simulink model "Bramki_zad1_4"  (R2025a)
settings: Solver=VariableStepAuto  StopTime=inf
libraries: visiontextngfix x1
settings Model: Creator=PM  LastModifiedBy=ai
settings SFSimCC: SimGPUStackLimitPerThread=51200  SimGPUMallocThreshold=200
settings RTWCC: GPUStackLimitPerThread=51200  GPUMallocThreshold=200

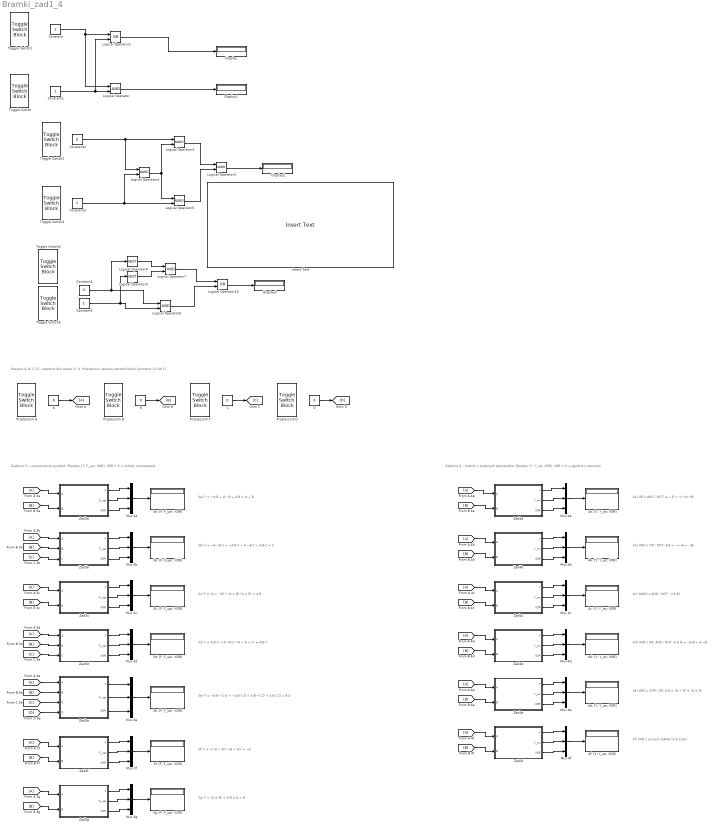
== system Bramki_zad1_4 ==
  note: Wejścia A, B, C, D – wspólne dla zadań 3 i 4. Przełącznik ustawia wartość bloku Constant (0 lub 1).
  note: 3a) F = ¬A·B + A·¬B + A·B = A + B
  note: 3b) F = ¬A·¬B·C + ¬A·B·C + A·¬B·C + A·B·C = C
  note: 3c) F = (A + ¬B)·(¬A + B)·(A + B) = A·B
  note: 3d) F = A·B·C·¬(A·¬B·C)·(A + B + C) = A·B·C
  note: 3e) F = ¬A·B·¬C·D + ¬A·B·C·D + A·B·¬C·D + A·B·C·D = B·D
  note: 3f) F = ¬((A + B)·(¬B + A)) = ¬A
  note: 3g) F = (A ⊕ B) + A·B = A + B
  note: 4a) OR z AND i NOT: A + B = ¬(¬A·¬B)
  note: 4b) AND z OR i NOT: A·B = ¬(¬A + ¬B)
  note: 4c) NAND z AND i NOT: ¬(A·B)
  note: 4d) XOR z OR, AND i NOT: A ⊕ B = ¬A·B + A·¬B
  note: 4e) AND z XOR i OR: A·B = (A + B) ⊕ (A ⊕ B)
  note: 4f) XOR z samych NAND (4 bramki)
  note: Zadanie 3 – upraszczanie wyrażeń. Display: [F; F_upr; XOR], XOR = 0 → układy równoważne
  note: Zadanie 4 – bramki z podanych elementów. Display: [Y; Y_wz; XOR], XOR = 0 → zgodne z wzorcem
  3a: [F; F_upr; XOR] : Display
  3b: [F; F_upr; XOR] : Display
  3c: [F; F_upr; XOR] : Display
  3d: [F; F_upr; XOR] : Display
  3e: [F; F_upr; XOR] : Display
  3f: [F; F_upr; XOR] : Display
  3g: [F; F_upr; XOR] : Display
  4a: [Y; Y_wz; XOR] : Display
  4b: [Y; Y_wz; XOR] : Display
  4c: [Y; Y_wz; XOR] : Display
  4d: [Y; Y_wz; XOR] : Display
  4e: [Y; Y_wz; XOR] : Display
  4f: [Y; Y_wz; XOR] : Display
  A : Constant  Value=0  OutDataTypeStr=boolean  SampleTime=0.1
  B : Constant  Value=0  OutDataTypeStr=boolean  SampleTime=0.1
  C : Constant  Value=0  OutDataTypeStr=boolean  SampleTime=0.1
  Constant{,1,3,5} (4 alike) : Constant
  Constant2 : Constant  Value=0
  Constant4 : Constant  Value=0
  D : Constant  Value=0  OutDataTypeStr=boolean  SampleTime=0.1
  Display{,1..3} (4 alike) : Display
  From A 3a : From
  From A 3b : From
  From A 3c : From
  From A 3d : From
  From A 3e : From
  From A 3f : From
  From A 3g : From
  From A 4a : From
  From A 4b : From
  From A 4c : From
  From A 4d : From
  From A 4e : From
  From A 4f : From
  Goto A : Goto
  Insert Text : visiontextngfix/Insert Text  inputType=Obsolete  theText='TO JEST TO SAMO wooooooooow'  getTextLocFrom=Specify via dialog  textLoc=[1 1]  getTextColorFrom=Specify via dialog  textColor=[0 0 0]  getTextIntensityFrom=Specify via dialog  textIntensity=0  getTextOpacityFrom=Specify via dialog  textOpacity=1.0  dummyVar2=0  dummyVar3=0  dummyVar4=0  imagePorts=One multidimensional signal  isInputTransposed=off  fontFace=LucidaSansRegular  dummyVar1=0  blockFontSize=12  antiAliased=on
  Logical Operator : Logic  AllPortsSameDT=off  OutDataTypeStr=boolean
  Logical Operator1 : Logic  Operator=OR  AllPortsSameDT=off  OutDataTypeStr=boolean
  Logical Operator10 : Logic  Operator=OR  AllPortsSameDT=off  OutDataTypeStr=boolean
  Logical Operator{2..5} (4 alike) : Logic  Operator=NAND  AllPortsSameDT=off  OutDataTypeStr=boolean
  Logical Operator6 : Logic  AllPortsSameDT=off  OutDataTypeStr=boolean
  Logical Operator7 : Logic  AllPortsSameDT=off  OutDataTypeStr=boolean
  Logical Operator8 : Logic  Operator=NOT  AllPortsSameDT=off  OutDataTypeStr=boolean
  Logical Operator9 : Logic  Operator=NOT  AllPortsSameDT=off  OutDataTypeStr=boolean
  Mux 3a : Mux  Inputs=3
  Mux 3b : Mux  Inputs=3
  Mux 3c : Mux  Inputs=3
  Mux 3d : Mux  Inputs=3
  Mux 3e : Mux  Inputs=3
  Mux 3f : Mux  Inputs=3
  Mux 3g : Mux  Inputs=3
  Mux 4a : Mux  Inputs=3
  Mux 4b : Mux  Inputs=3
  Mux 4c : Mux  Inputs=3
  Mux 4d : Mux  Inputs=3
  Mux 4e : Mux  Inputs=3
  Mux 4f : Mux  Inputs=3
  Przelacznik A : ToggleSwitchBlock
  Przelacznik B : ToggleSwitchBlock
  Przelacznik C : ToggleSwitchBlock
  Przelacznik D : ToggleSwitchBlock
  Toggle Switch{,1..5} (6 alike) : ToggleSwitchBlock
  Zad3a : Subsystem
  Zad3b : Subsystem
  Zad3c : Subsystem
  Zad3d : Subsystem
  Zad3e : Subsystem
  Zad3f : Subsystem
  Zad3g : Subsystem
  Zad4a : Subsystem
  Zad4b : Subsystem
  Zad4c : Subsystem
  Zad4d : Subsystem
  Zad4e : Subsystem
  Zad4f : Subsystem
  wires:
  Constant/1 -> Logical Operator/1, Logical Operator1/1
  Constant1/1 -> Logical Operator/2, Logical Operator1/2
  Logical Operator1/1 -> Display/1
  Logical Operator/1 -> Display1/1
  Logical Operator2/1 -> Logical Operator3/1
  Logical Operator5/1 -> Logical Operator3/2
  Logical Operator4/1 -> Logical Operator5/1, Logical Operator2/2
  Constant2/1 -> Logical Operator4/1, Logical Operator2/1
  Constant3/1 -> Logical Operator4/2, Logical Operator5/2
  Logical Operator3/1 -> Display2/1
  Logical Operator7/1 -> Logical Operator10/1
  Logical Operator6/1 -> Logical Operator10/2
  Logical Operator10/1 -> Display3/1
  Logical Operator8/1 -> Logical Operator7/1
  Logical Operator9/1 -> Logical Operator7/2
  Constant5/1 -> Logical Operator9/1, Logical Operator6/2
  Constant4/1 -> Logical Operator8/1, Logical Operator6/1
  A/1 -> Goto A/1
  B/1 -> [B]
  C/1 -> [C]
  D/1 -> [D]
  From A 3a/1 -> Zad3a/1(A)
  [B] -> Zad3a/2(B)
  Zad3a/1(F) -> Mux 3a/1
  Zad3a/2(F_upr) -> Mux 3a/2
  Zad3a/3(XOR) -> Mux 3a/3
  Mux 3a/1 -> 3a: [F; F_upr; XOR]/1
  From A 3b/1 -> Zad3b/1(A)
  [B] -> Zad3b/2(B)
  [C] -> Zad3b/3(C)
  Zad3b/1(F) -> Mux 3b/1
  Zad3b/2(F_upr) -> Mux 3b/2
  Zad3b/3(XOR) -> Mux 3b/3
  Mux 3b/1 -> 3b: [F; F_upr; XOR]/1
  From A 3c/1 -> Zad3c/1(A)
  [B] -> Zad3c/2(B)
  Zad3c/1(F) -> Mux 3c/1
  Zad3c/2(F_upr) -> Mux 3c/2
  Zad3c/3(XOR) -> Mux 3c/3
  Mux 3c/1 -> 3c: [F; F_upr; XOR]/1
  From A 3d/1 -> Zad3d/1(A)
  [B] -> Zad3d/2(B)
  [C] -> Zad3d/3(C)
  Zad3d/1(F) -> Mux 3d/1
  Zad3d/2(F_upr) -> Mux 3d/2
  Zad3d/3(XOR) -> Mux 3d/3
  Mux 3d/1 -> 3d: [F; F_upr; XOR]/1
  From A 3e/1 -> Zad3e/1(A)
  [B] -> Zad3e/2(B)
  [C] -> Zad3e/3(C)
  [D] -> Zad3e/4(D)
  Zad3e/1(F) -> Mux 3e/1
  Zad3e/2(F_upr) -> Mux 3e/2
  Zad3e/3(XOR) -> Mux 3e/3
  Mux 3e/1 -> 3e: [F; F_upr; XOR]/1
  From A 3f/1 -> Zad3f/1(A)
  [B] -> Zad3f/2(B)
  Zad3f/1(F) -> Mux 3f/1
  Zad3f/2(F_upr) -> Mux 3f/2
  Zad3f/3(XOR) -> Mux 3f/3
  Mux 3f/1 -> 3f: [F; F_upr; XOR]/1
  From A 3g/1 -> Zad3g/1(A)
  [B] -> Zad3g/2(B)
  Zad3g/1(F) -> Mux 3g/1
  Zad3g/2(F_upr) -> Mux 3g/2
  Zad3g/3(XOR) -> Mux 3g/3
  Mux 3g/1 -> 3g: [F; F_upr; XOR]/1
  From A 4a/1 -> Zad4a/1(A)
  [B] -> Zad4a/2(B)
  Zad4a/1(Y) -> Mux 4a/1
  Zad4a/2(Y_wz) -> Mux 4a/2
  Zad4a/3(XOR) -> Mux 4a/3
  Mux 4a/1 -> 4a: [Y; Y_wz; XOR]/1
  From A 4b/1 -> Zad4b/1(A)
  [B] -> Zad4b/2(B)
  Zad4b/1(Y) -> Mux 4b/1
  Zad4b/2(Y_wz) -> Mux 4b/2
  Zad4b/3(XOR) -> Mux 4b/3
  Mux 4b/1 -> 4b: [Y; Y_wz; XOR]/1
  From A 4c/1 -> Zad4c/1(A)
  [B] -> Zad4c/2(B)
  Zad4c/1(Y) -> Mux 4c/1
  Zad4c/2(Y_wz) -> Mux 4c/2
  Zad4c/3(XOR) -> Mux 4c/3
  Mux 4c/1 -> 4c: [Y; Y_wz; XOR]/1
  From A 4d/1 -> Zad4d/1(A)
  [B] -> Zad4d/2(B)
  Zad4d/1(Y) -> Mux 4d/1
  Zad4d/2(Y_wz) -> Mux 4d/2
  Zad4d/3(XOR) -> Mux 4d/3
  Mux 4d/1 -> 4d: [Y; Y_wz; XOR]/1
  From A 4e/1 -> Zad4e/1(A)
  [B] -> Zad4e/2(B)
  Zad4e/1(Y) -> Mux 4e/1
  Zad4e/2(Y_wz) -> Mux 4e/2
  Zad4e/3(XOR) -> Mux 4e/3
  Mux 4e/1 -> 4e: [Y; Y_wz; XOR]/1
  From A 4f/1 -> Zad4f/1(A)
  [B] -> Zad4f/2(B)
  Zad4f/1(Y) -> Mux 4f/1
  Zad4f/2(Y_wz) -> Mux 4f/2
  Zad4f/3(XOR) -> Mux 4f/3
  Mux 4f/1 -> 4f: [Y; Y_wz; XOR]/1

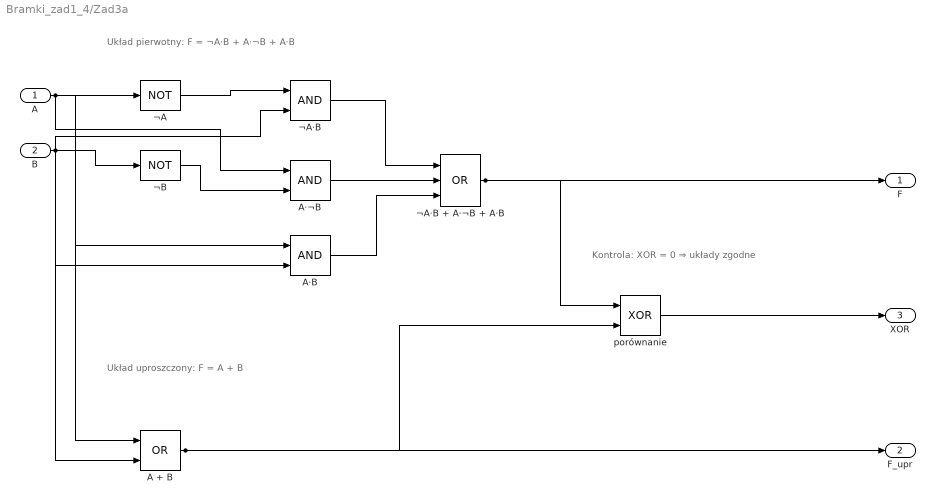
== system Bramki_zad1_4/Zad3a ==
  note: Układ pierwotny: F = ¬A·B + A·¬B + A·B
  note: Układ uproszczony: F = A + B
  note: Kontrola: XOR = 0 ⇒ układy zgodne
  A : Inport
  B : Inport  Port=2
  A + B : Logic  Operator=OR  IconShape=distinctive  AllPortsSameDT=off  OutDataTypeStr=boolean
  A·B : Logic  IconShape=distinctive  AllPortsSameDT=off  OutDataTypeStr=boolean
  A·¬B : Logic  IconShape=distinctive  AllPortsSameDT=off  OutDataTypeStr=boolean
  porównanie : Logic  Operator=XOR  IconShape=distinctive  AllPortsSameDT=off  OutDataTypeStr=boolean
  ¬A : Logic  Operator=NOT  Inputs=1  IconShape=distinctive  AllPortsSameDT=off  OutDataTypeStr=boolean
  ¬A·B : Logic  IconShape=distinctive  AllPortsSameDT=off  OutDataTypeStr=boolean
  ¬A·B + A·¬B + A·B : Logic  Operator=OR  Inputs=3  IconShape=distinctive  AllPortsSameDT=off  OutDataTypeStr=boolean
  ¬B : Logic  Operator=NOT  Inputs=1  IconShape=distinctive  AllPortsSameDT=off  OutDataTypeStr=boolean
  F : Outport
  F_upr : Outport  Port=2
  XOR : Outport  Port=3
  wires:
  A/1 -> ¬A/1, A·¬B/1, A·B/1, A + B/1
  B/1 -> ¬B/1, ¬A·B/2, A·B/2, A + B/2
  ¬A/1 -> ¬A·B/1
  ¬B/1 -> A·¬B/2
  ¬A·B/1 -> ¬A·B + A·¬B + A·B/1
  A·¬B/1 -> ¬A·B + A·¬B + A·B/2
  A·B/1 -> ¬A·B + A·¬B + A·B/3
  ¬A·B + A·¬B + A·B/1 -> porównanie/1, F/1
  A + B/1 -> porównanie/2, F_upr/1
  porównanie/1 -> XOR/1

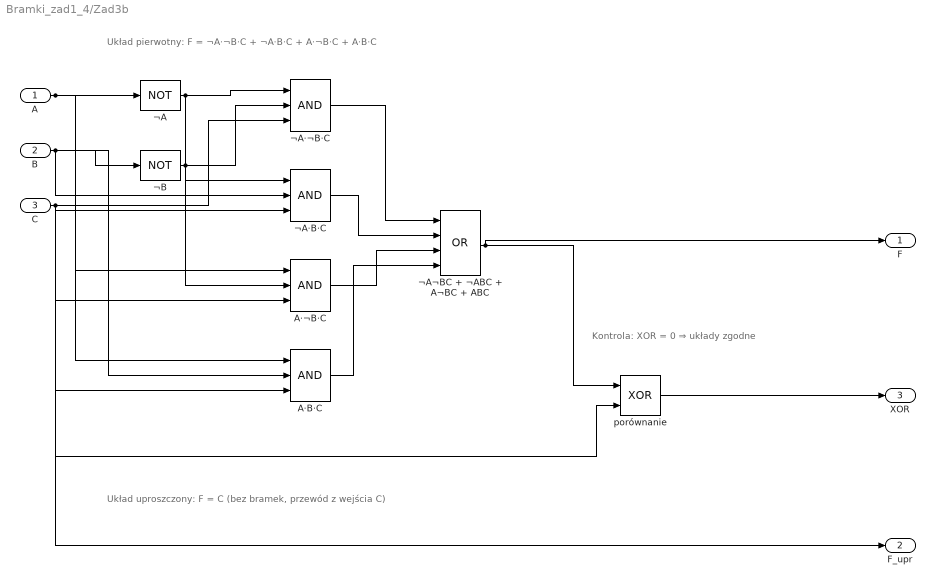
== system Bramki_zad1_4/Zad3b ==
  note: Układ pierwotny: F = ¬A·¬B·C + ¬A·B·C + A·¬B·C + A·B·C
  note: Układ uproszczony: F = C (bez bramek, przewód z wejścia C)
  note: Kontrola: XOR = 0 ⇒ układy zgodne
  A : Inport
  B : Inport  Port=2
  C : Inport  Port=3
  A·B·C : Logic  Inputs=3  IconShape=distinctive  AllPortsSameDT=off  OutDataTypeStr=boolean
  A·¬B·C : Logic  Inputs=3  IconShape=distinctive  AllPortsSameDT=off  OutDataTypeStr=boolean
  porównanie : Logic  Operator=XOR  IconShape=distinctive  AllPortsSameDT=off  OutDataTypeStr=boolean
  ¬A : Logic  Operator=NOT  Inputs=1  IconShape=distinctive  AllPortsSameDT=off  OutDataTypeStr=boolean
  ¬A¬BC + ¬ABC + A¬BC + ABC : Logic  Operator=OR  Inputs=4  IconShape=distinctive  AllPortsSameDT=off  OutDataTypeStr=boolean
  ¬A·B·C : Logic  Inputs=3  IconShape=distinctive  AllPortsSameDT=off  OutDataTypeStr=boolean
  ¬A·¬B·C : Logic  Inputs=3  IconShape=distinctive  AllPortsSameDT=off  OutDataTypeStr=boolean
  ¬B : Logic  Operator=NOT  Inputs=1  IconShape=distinctive  AllPortsSameDT=off  OutDataTypeStr=boolean
  F : Outport
  F_upr : Outport  Port=2
  XOR : Outport  Port=3
  wires:
  A/1 -> ¬A/1, A·¬B·C/1, A·B·C/1
  B/1 -> ¬B/1, ¬A·B·C/2, A·B·C/2
  ¬A/1 -> ¬A·¬B·C/1, ¬A·B·C/1
  ¬B/1 -> ¬A·¬B·C/2, A·¬B·C/2
  C/1 -> ¬A·¬B·C/3, ¬A·B·C/3, A·¬B·C/3, A·B·C/3, porównanie/2, F_upr/1
  ¬A·¬B·C/1 -> ¬A¬BC + ¬ABC + A¬BC + ABC/1
  ¬A·B·C/1 -> ¬A¬BC + ¬ABC + A¬BC + ABC/2
  A·¬B·C/1 -> ¬A¬BC + ¬ABC + A¬BC + ABC/3
  A·B·C/1 -> ¬A¬BC + ¬ABC + A¬BC + ABC/4
  ¬A¬BC + ¬ABC + A¬BC + ABC/1 -> porównanie/1, F/1
  porównanie/1 -> XOR/1

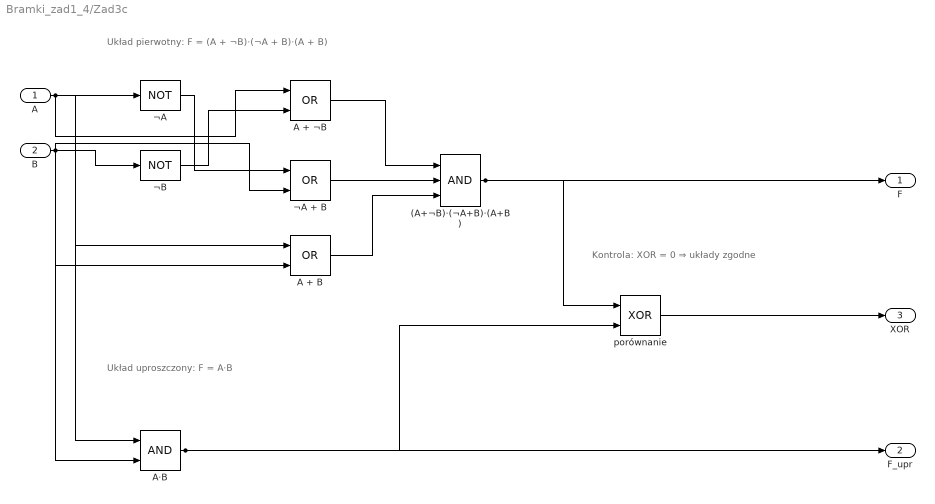
== system Bramki_zad1_4/Zad3c ==
  note: Układ pierwotny: F = (A + ¬B)·(¬A + B)·(A + B)
  note: Układ uproszczony: F = A·B
  note: Kontrola: XOR = 0 ⇒ układy zgodne
  A : Inport
  B : Inport  Port=2
  (A+¬B)·(¬A+B)·(A+B) : Logic  Inputs=3  IconShape=distinctive  AllPortsSameDT=off  OutDataTypeStr=boolean
  A + B : Logic  Operator=OR  IconShape=distinctive  AllPortsSameDT=off  OutDataTypeStr=boolean
  A + ¬B : Logic  Operator=OR  IconShape=distinctive  AllPortsSameDT=off  OutDataTypeStr=boolean
  A·B : Logic  IconShape=distinctive  AllPortsSameDT=off  OutDataTypeStr=boolean
  porównanie : Logic  Operator=XOR  IconShape=distinctive  AllPortsSameDT=off  OutDataTypeStr=boolean
  ¬A : Logic  Operator=NOT  Inputs=1  IconShape=distinctive  AllPortsSameDT=off  OutDataTypeStr=boolean
  ¬A + B : Logic  Operator=OR  IconShape=distinctive  AllPortsSameDT=off  OutDataTypeStr=boolean
  ¬B : Logic  Operator=NOT  Inputs=1  IconShape=distinctive  AllPortsSameDT=off  OutDataTypeStr=boolean
  F : Outport
  F_upr : Outport  Port=2
  XOR : Outport  Port=3
  wires:
  A/1 -> ¬A/1, A + ¬B/1, A + B/1, A·B/1
  B/1 -> ¬B/1, ¬A + B/2, A + B/2, A·B/2
  ¬B/1 -> A + ¬B/2
  ¬A/1 -> ¬A + B/1
  A + ¬B/1 -> (A+¬B)·(¬A+B)·(A+B)/1
  ¬A + B/1 -> (A+¬B)·(¬A+B)·(A+B)/2
  A + B/1 -> (A+¬B)·(¬A+B)·(A+B)/3
  (A+¬B)·(¬A+B)·(A+B)/1 -> porównanie/1, F/1
  A·B/1 -> porównanie/2, F_upr/1
  porównanie/1 -> XOR/1

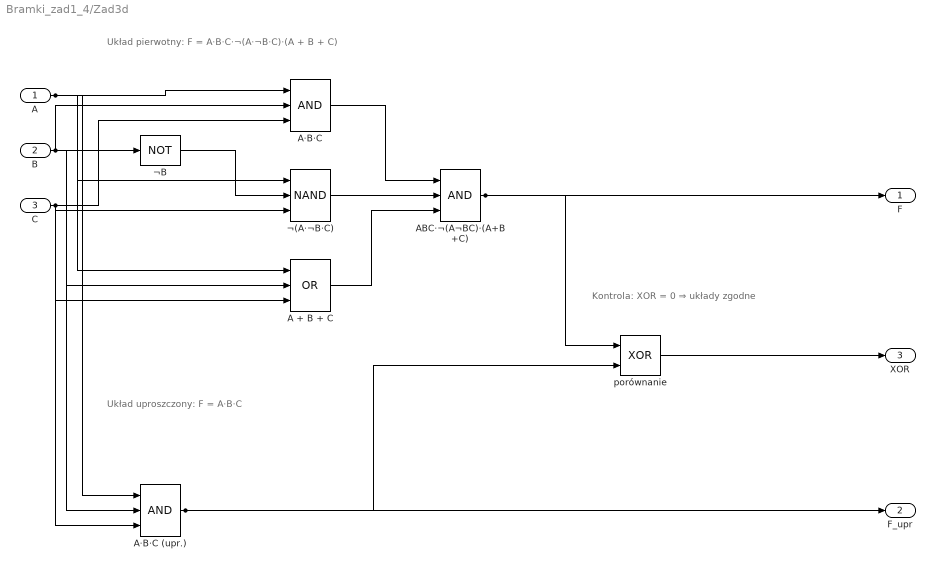
== system Bramki_zad1_4/Zad3d ==
  note: Układ pierwotny: F = A·B·C·¬(A·¬B·C)·(A + B + C)
  note: Układ uproszczony: F = A·B·C
  note: Kontrola: XOR = 0 ⇒ układy zgodne
  A : Inport
  B : Inport  Port=2
  C : Inport  Port=3
  A + B + C : Logic  Operator=OR  Inputs=3  IconShape=distinctive  AllPortsSameDT=off  OutDataTypeStr=boolean
  ABC·¬(A¬BC)·(A+B+C) : Logic  Inputs=3  IconShape=distinctive  AllPortsSameDT=off  OutDataTypeStr=boolean
  A·B·C : Logic  Inputs=3  IconShape=distinctive  AllPortsSameDT=off  OutDataTypeStr=boolean
  A·B·C (upr.) : Logic  Inputs=3  IconShape=distinctive  AllPortsSameDT=off  OutDataTypeStr=boolean
  porównanie : Logic  Operator=XOR  IconShape=distinctive  AllPortsSameDT=off  OutDataTypeStr=boolean
  ¬(A·¬B·C) : Logic  Operator=NAND  Inputs=3  IconShape=distinctive  AllPortsSameDT=off  OutDataTypeStr=boolean
  ¬B : Logic  Operator=NOT  Inputs=1  IconShape=distinctive  AllPortsSameDT=off  OutDataTypeStr=boolean
  F : Outport
  F_upr : Outport  Port=2
  XOR : Outport  Port=3
  wires:
  B/1 -> ¬B/1, A·B·C/2, A + B + C/2, A·B·C (upr.)/2
  A/1 -> A·B·C/1, ¬(A·¬B·C)/1, A + B + C/1, A·B·C (upr.)/1
  C/1 -> A·B·C/3, ¬(A·¬B·C)/3, A + B + C/3, A·B·C (upr.)/3
  ¬B/1 -> ¬(A·¬B·C)/2
  A·B·C/1 -> ABC·¬(A¬BC)·(A+B+C)/1
  ¬(A·¬B·C)/1 -> ABC·¬(A¬BC)·(A+B+C)/2
  A + B + C/1 -> ABC·¬(A¬BC)·(A+B+C)/3
  ABC·¬(A¬BC)·(A+B+C)/1 -> porównanie/1, F/1
  A·B·C (upr.)/1 -> porównanie/2, F_upr/1
  porównanie/1 -> XOR/1

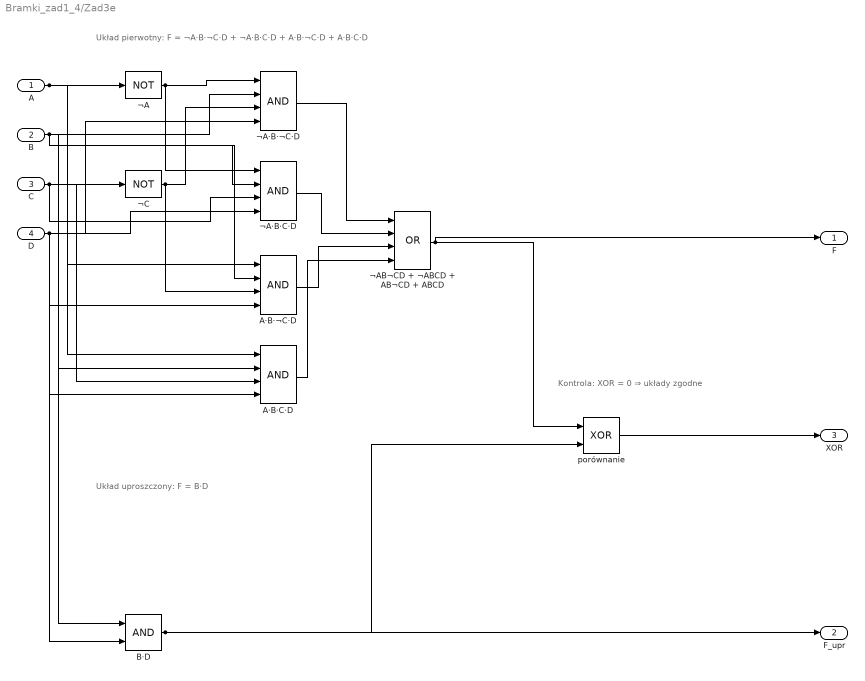
== system Bramki_zad1_4/Zad3e ==
  note: Układ pierwotny: F = ¬A·B·¬C·D + ¬A·B·C·D + A·B·¬C·D + A·B·C·D
  note: Układ uproszczony: F = B·D
  note: Kontrola: XOR = 0 ⇒ układy zgodne
  A : Inport
  B : Inport  Port=2
  C : Inport  Port=3
  D : Inport  Port=4
  A·B·C·D : Logic  Inputs=4  IconShape=distinctive  AllPortsSameDT=off  OutDataTypeStr=boolean
  A·B·¬C·D : Logic  Inputs=4  IconShape=distinctive  AllPortsSameDT=off  OutDataTypeStr=boolean
  B·D : Logic  IconShape=distinctive  AllPortsSameDT=off  OutDataTypeStr=boolean
  porównanie : Logic  Operator=XOR  IconShape=distinctive  AllPortsSameDT=off  OutDataTypeStr=boolean
  ¬A : Logic  Operator=NOT  Inputs=1  IconShape=distinctive  AllPortsSameDT=off  OutDataTypeStr=boolean
  ¬AB¬CD + ¬ABCD + AB¬CD + ABCD : Logic  Operator=OR  Inputs=4  IconShape=distinctive  AllPortsSameDT=off  OutDataTypeStr=boolean
  ¬A·B·C·D : Logic  Inputs=4  IconShape=distinctive  AllPortsSameDT=off  OutDataTypeStr=boolean
  ¬A·B·¬C·D : Logic  Inputs=4  IconShape=distinctive  AllPortsSameDT=off  OutDataTypeStr=boolean
  ¬C : Logic  Operator=NOT  Inputs=1  IconShape=distinctive  AllPortsSameDT=off  OutDataTypeStr=boolean
  F : Outport
  F_upr : Outport  Port=2
  XOR : Outport  Port=3
  wires:
  A/1 -> ¬A/1, A·B·¬C·D/1, A·B·C·D/1
  C/1 -> ¬C/1, ¬A·B·C·D/3, A·B·C·D/3
  ¬A/1 -> ¬A·B·¬C·D/1, ¬A·B·C·D/1
  B/1 -> ¬A·B·¬C·D/2, ¬A·B·C·D/2, A·B·¬C·D/2, A·B·C·D/2, B·D/1
  ¬C/1 -> ¬A·B·¬C·D/3, A·B·¬C·D/3
  D/1 -> ¬A·B·¬C·D/4, ¬A·B·C·D/4, A·B·¬C·D/4, A·B·C·D/4, B·D/2
  ¬A·B·¬C·D/1 -> ¬AB¬CD + ¬ABCD + AB¬CD + ABCD/1
  ¬A·B·C·D/1 -> ¬AB¬CD + ¬ABCD + AB¬CD + ABCD/2
  A·B·¬C·D/1 -> ¬AB¬CD + ¬ABCD + AB¬CD + ABCD/3
  A·B·C·D/1 -> ¬AB¬CD + ¬ABCD + AB¬CD + ABCD/4
  ¬AB¬CD + ¬ABCD + AB¬CD + ABCD/1 -> porównanie/1, F/1
  B·D/1 -> porównanie/2, F_upr/1
  porównanie/1 -> XOR/1

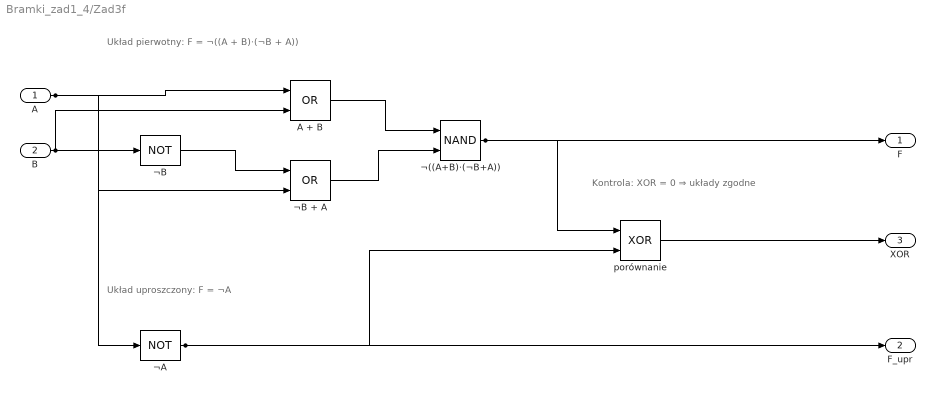
== system Bramki_zad1_4/Zad3f ==
  note: Układ pierwotny: F = ¬((A + B)·(¬B + A))
  note: Układ uproszczony: F = ¬A
  note: Kontrola: XOR = 0 ⇒ układy zgodne
  A : Inport
  B : Inport  Port=2
  A + B : Logic  Operator=OR  IconShape=distinctive  AllPortsSameDT=off  OutDataTypeStr=boolean
  porównanie : Logic  Operator=XOR  IconShape=distinctive  AllPortsSameDT=off  OutDataTypeStr=boolean
  ¬((A+B)·(¬B+A)) : Logic  Operator=NAND  IconShape=distinctive  AllPortsSameDT=off  OutDataTypeStr=boolean
  ¬A : Logic  Operator=NOT  Inputs=1  IconShape=distinctive  AllPortsSameDT=off  OutDataTypeStr=boolean
  ¬B : Logic  Operator=NOT  Inputs=1  IconShape=distinctive  AllPortsSameDT=off  OutDataTypeStr=boolean
  ¬B + A : Logic  Operator=OR  IconShape=distinctive  AllPortsSameDT=off  OutDataTypeStr=boolean
  F : Outport
  F_upr : Outport  Port=2
  XOR : Outport  Port=3
  wires:
  B/1 -> ¬B/1, A + B/2
  A/1 -> A + B/1, ¬B + A/2, ¬A/1
  ¬B/1 -> ¬B + A/1
  A + B/1 -> ¬((A+B)·(¬B+A))/1
  ¬B + A/1 -> ¬((A+B)·(¬B+A))/2
  ¬((A+B)·(¬B+A))/1 -> porównanie/1, F/1
  ¬A/1 -> porównanie/2, F_upr/1
  porównanie/1 -> XOR/1

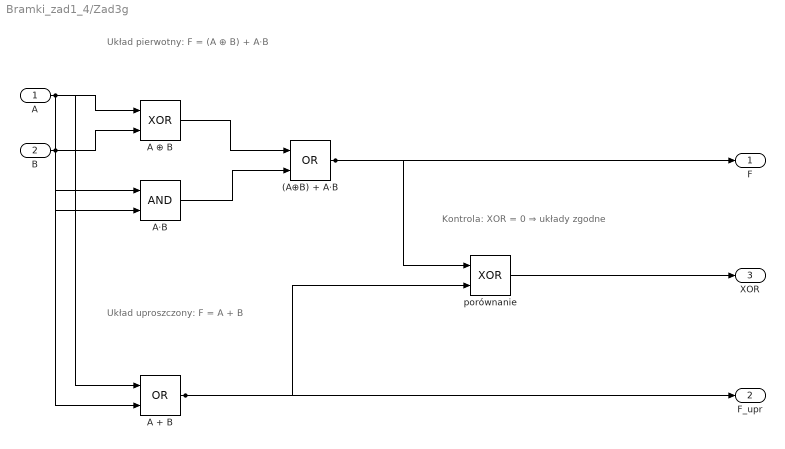
== system Bramki_zad1_4/Zad3g ==
  note: Układ pierwotny: F = (A ⊕ B) + A·B
  note: Układ uproszczony: F = A + B
  note: Kontrola: XOR = 0 ⇒ układy zgodne
  A : Inport
  B : Inport  Port=2
  (A⊕B) + A·B : Logic  Operator=OR  IconShape=distinctive  AllPortsSameDT=off  OutDataTypeStr=boolean
  A + B : Logic  Operator=OR  IconShape=distinctive  AllPortsSameDT=off  OutDataTypeStr=boolean
  A ⊕ B : Logic  Operator=XOR  IconShape=distinctive  AllPortsSameDT=off  OutDataTypeStr=boolean
  A·B : Logic  IconShape=distinctive  AllPortsSameDT=off  OutDataTypeStr=boolean
  porównanie : Logic  Operator=XOR  IconShape=distinctive  AllPortsSameDT=off  OutDataTypeStr=boolean
  F : Outport
  F_upr : Outport  Port=2
  XOR : Outport  Port=3
  wires:
  A/1 -> A ⊕ B/1, A·B/1, A + B/1
  B/1 -> A ⊕ B/2, A·B/2, A + B/2
  A ⊕ B/1 -> (A⊕B) + A·B/1
  A·B/1 -> (A⊕B) + A·B/2
  (A⊕B) + A·B/1 -> porównanie/1, F/1
  A + B/1 -> porównanie/2, F_upr/1
  porównanie/1 -> XOR/1

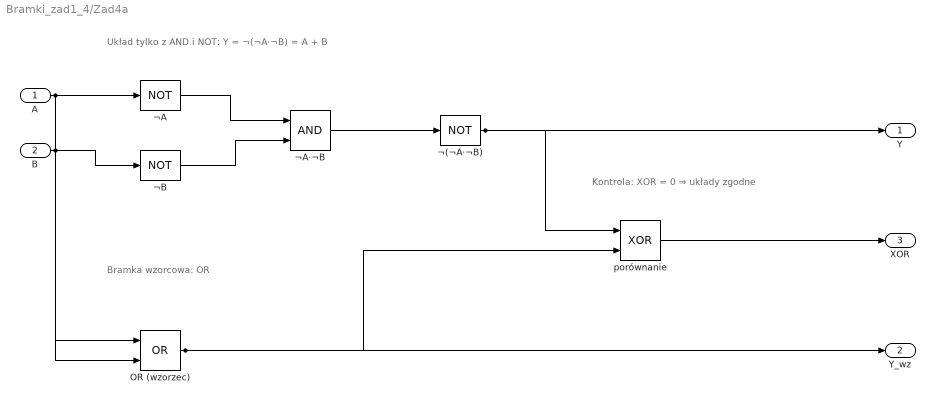
== system Bramki_zad1_4/Zad4a ==
  note: Układ tylko z AND i NOT: Y = ¬(¬A·¬B) = A + B
  note: Bramka wzorcowa: OR
  note: Kontrola: XOR = 0 ⇒ układy zgodne
  A : Inport
  B : Inport  Port=2
  OR (wzorzec) : Logic  Operator=OR  IconShape=distinctive  AllPortsSameDT=off  OutDataTypeStr=boolean
  porównanie : Logic  Operator=XOR  IconShape=distinctive  AllPortsSameDT=off  OutDataTypeStr=boolean
  ¬(¬A·¬B) : Logic  Operator=NOT  Inputs=1  IconShape=distinctive  AllPortsSameDT=off  OutDataTypeStr=boolean
  ¬A : Logic  Operator=NOT  Inputs=1  IconShape=distinctive  AllPortsSameDT=off  OutDataTypeStr=boolean
  ¬A·¬B : Logic  IconShape=distinctive  AllPortsSameDT=off  OutDataTypeStr=boolean
  ¬B : Logic  Operator=NOT  Inputs=1  IconShape=distinctive  AllPortsSameDT=off  OutDataTypeStr=boolean
  Y : Outport
  Y_wz : Outport  Port=2
  XOR : Outport  Port=3
  wires:
  A/1 -> ¬A/1, OR (wzorzec)/1
  B/1 -> ¬B/1, OR (wzorzec)/2
  ¬A/1 -> ¬A·¬B/1
  ¬B/1 -> ¬A·¬B/2
  ¬A·¬B/1 -> ¬(¬A·¬B)/1
  ¬(¬A·¬B)/1 -> porównanie/1, Y/1
  OR (wzorzec)/1 -> porównanie/2, Y_wz/1
  porównanie/1 -> XOR/1

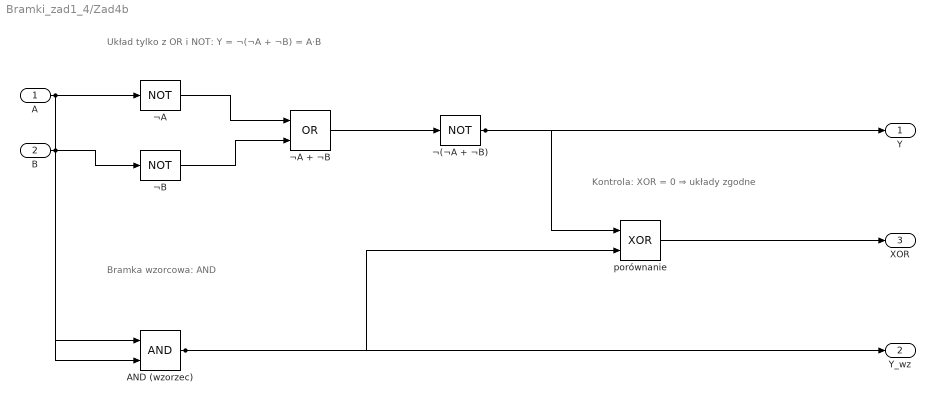
== system Bramki_zad1_4/Zad4b ==
  note: Układ tylko z OR i NOT: Y = ¬(¬A + ¬B) = A·B
  note: Bramka wzorcowa: AND
  note: Kontrola: XOR = 0 ⇒ układy zgodne
  A : Inport
  B : Inport  Port=2
  AND (wzorzec) : Logic  IconShape=distinctive  AllPortsSameDT=off  OutDataTypeStr=boolean
  porównanie : Logic  Operator=XOR  IconShape=distinctive  AllPortsSameDT=off  OutDataTypeStr=boolean
  ¬(¬A + ¬B) : Logic  Operator=NOT  Inputs=1  IconShape=distinctive  AllPortsSameDT=off  OutDataTypeStr=boolean
  ¬A : Logic  Operator=NOT  Inputs=1  IconShape=distinctive  AllPortsSameDT=off  OutDataTypeStr=boolean
  ¬A + ¬B : Logic  Operator=OR  IconShape=distinctive  AllPortsSameDT=off  OutDataTypeStr=boolean
  ¬B : Logic  Operator=NOT  Inputs=1  IconShape=distinctive  AllPortsSameDT=off  OutDataTypeStr=boolean
  Y : Outport
  Y_wz : Outport  Port=2
  XOR : Outport  Port=3
  wires:
  A/1 -> ¬A/1, AND (wzorzec)/1
  B/1 -> ¬B/1, AND (wzorzec)/2
  ¬A/1 -> ¬A + ¬B/1
  ¬B/1 -> ¬A + ¬B/2
  ¬A + ¬B/1 -> ¬(¬A + ¬B)/1
  ¬(¬A + ¬B)/1 -> porównanie/1, Y/1
  AND (wzorzec)/1 -> porównanie/2, Y_wz/1
  porównanie/1 -> XOR/1

== system Bramki_zad1_4/Zad4c ==
  note: Układ tylko z AND i NOT: Y = ¬(A·B)
  note: Bramka wzorcowa: NAND
  note: Kontrola: XOR = 0 ⇒ układy zgodne
  A : Inport
  B : Inport  Port=2
  A·B : Logic  IconShape=distinctive  AllPortsSameDT=off  OutDataTypeStr=boolean
  NAND (wzorzec) : Logic  Operator=NAND  IconShape=distinctive  AllPortsSameDT=off  OutDataTypeStr=boolean
  porównanie : Logic  Operator=XOR  IconShape=distinctive  AllPortsSameDT=off  OutDataTypeStr=boolean
  ¬(A·B) : Logic  Operator=NOT  Inputs=1  IconShape=distinctive  AllPortsSameDT=off  OutDataTypeStr=boolean
  Y : Outport
  Y_wz : Outport  Port=2
  XOR : Outport  Port=3
  wires:
  A/1 -> A·B/1, NAND (wzorzec)/1
  B/1 -> A·B/2, NAND (wzorzec)/2
  A·B/1 -> ¬(A·B)/1
  ¬(A·B)/1 -> porównanie/1, Y/1
  NAND (wzorzec)/1 -> porównanie/2, Y_wz/1
  porównanie/1 -> XOR/1

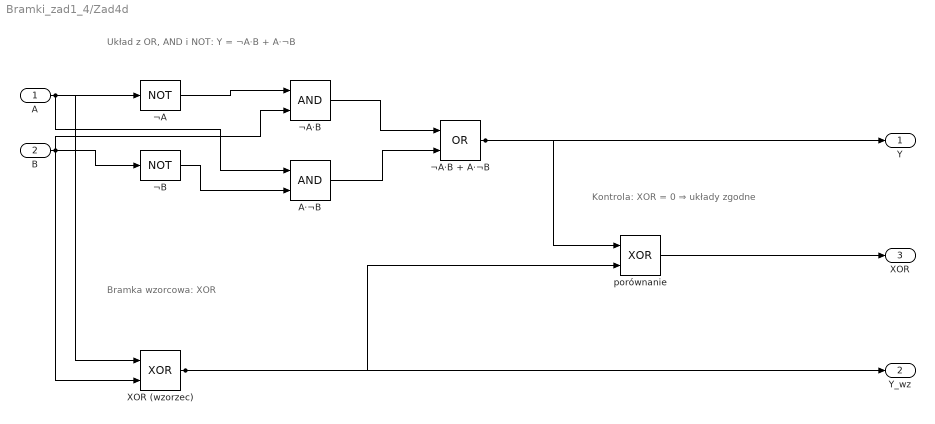
== system Bramki_zad1_4/Zad4d ==
  note: Układ z OR, AND i NOT: Y = ¬A·B + A·¬B
  note: Bramka wzorcowa: XOR
  note: Kontrola: XOR = 0 ⇒ układy zgodne
  A : Inport
  B : Inport  Port=2
  A·¬B : Logic  IconShape=distinctive  AllPortsSameDT=off  OutDataTypeStr=boolean
  XOR (wzorzec) : Logic  Operator=XOR  IconShape=distinctive  AllPortsSameDT=off  OutDataTypeStr=boolean
  porównanie : Logic  Operator=XOR  IconShape=distinctive  AllPortsSameDT=off  OutDataTypeStr=boolean
  ¬A : Logic  Operator=NOT  Inputs=1  IconShape=distinctive  AllPortsSameDT=off  OutDataTypeStr=boolean
  ¬A·B : Logic  IconShape=distinctive  AllPortsSameDT=off  OutDataTypeStr=boolean
  ¬A·B + A·¬B : Logic  Operator=OR  IconShape=distinctive  AllPortsSameDT=off  OutDataTypeStr=boolean
  ¬B : Logic  Operator=NOT  Inputs=1  IconShape=distinctive  AllPortsSameDT=off  OutDataTypeStr=boolean
  Y : Outport
  Y_wz : Outport  Port=2
  XOR : Outport  Port=3
  wires:
  A/1 -> ¬A/1, A·¬B/1, XOR (wzorzec)/1
  B/1 -> ¬B/1, ¬A·B/2, XOR (wzorzec)/2
  ¬A/1 -> ¬A·B/1
  ¬B/1 -> A·¬B/2
  ¬A·B/1 -> ¬A·B + A·¬B/1
  A·¬B/1 -> ¬A·B + A·¬B/2
  ¬A·B + A·¬B/1 -> porównanie/1, Y/1
  XOR (wzorzec)/1 -> porównanie/2, Y_wz/1
  porównanie/1 -> XOR/1

== system Bramki_zad1_4/Zad4e ==
  note: Układ tylko z XOR i OR: Y = (A + B) ⊕ (A ⊕ B) = A·B
  note: Bramka wzorcowa: AND
  note: Kontrola: XOR = 0 ⇒ układy zgodne
  A : Inport
  B : Inport  Port=2
  (A+B) ⊕ (A⊕B) : Logic  Operator=XOR  IconShape=distinctive  AllPortsSameDT=off  OutDataTypeStr=boolean
  A + B : Logic  Operator=OR  IconShape=distinctive  AllPortsSameDT=off  OutDataTypeStr=boolean
  A ⊕ B : Logic  Operator=XOR  IconShape=distinctive  AllPortsSameDT=off  OutDataTypeStr=boolean
  AND (wzorzec) : Logic  IconShape=distinctive  AllPortsSameDT=off  OutDataTypeStr=boolean
  porównanie : Logic  Operator=XOR  IconShape=distinctive  AllPortsSameDT=off  OutDataTypeStr=boolean
  Y : Outport
  Y_wz : Outport  Port=2
  XOR : Outport  Port=3
  wires:
  A/1 -> A + B/1, A ⊕ B/1, AND (wzorzec)/1
  B/1 -> A + B/2, A ⊕ B/2, AND (wzorzec)/2
  A + B/1 -> (A+B) ⊕ (A⊕B)/1
  A ⊕ B/1 -> (A+B) ⊕ (A⊕B)/2
  (A+B) ⊕ (A⊕B)/1 -> porównanie/1, Y/1
  AND (wzorzec)/1 -> porównanie/2, Y_wz/1
  porównanie/1 -> XOR/1

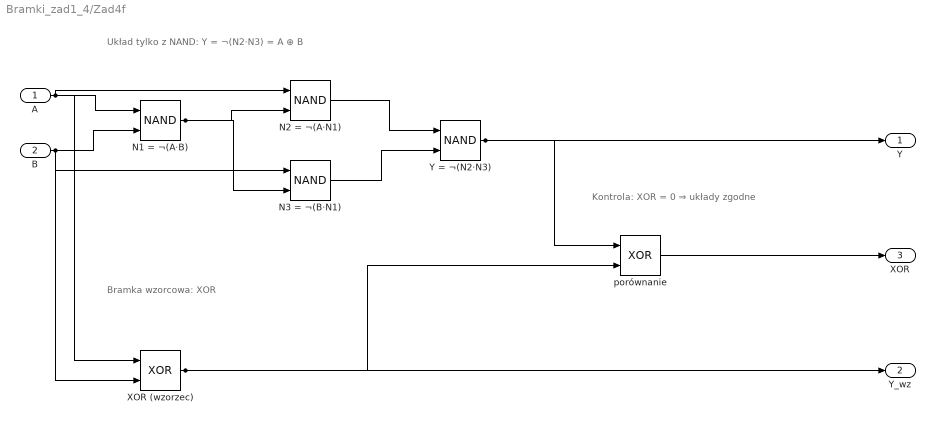
== system Bramki_zad1_4/Zad4f ==
  note: Układ tylko z NAND: Y = ¬(N2·N3) = A ⊕ B
  note: Bramka wzorcowa: XOR
  note: Kontrola: XOR = 0 ⇒ układy zgodne
  A : Inport
  B : Inport  Port=2
  N1 = ¬(A·B) : Logic  Operator=NAND  IconShape=distinctive  AllPortsSameDT=off  OutDataTypeStr=boolean
  N2 = ¬(A·N1) : Logic  Operator=NAND  IconShape=distinctive  AllPortsSameDT=off  OutDataTypeStr=boolean
  N3 = ¬(B·N1) : Logic  Operator=NAND  IconShape=distinctive  AllPortsSameDT=off  OutDataTypeStr=boolean
  XOR (wzorzec) : Logic  Operator=XOR  IconShape=distinctive  AllPortsSameDT=off  OutDataTypeStr=boolean
  Y = ¬(N2·N3) : Logic  Operator=NAND  IconShape=distinctive  AllPortsSameDT=off  OutDataTypeStr=boolean
  porównanie : Logic  Operator=XOR  IconShape=distinctive  AllPortsSameDT=off  OutDataTypeStr=boolean
  Y : Outport
  Y_wz : Outport  Port=2
  XOR : Outport  Port=3
  wires:
  A/1 -> N1 = ¬(A·B)/1, N2 = ¬(A·N1)/1, XOR (wzorzec)/1
  B/1 -> N1 = ¬(A·B)/2, N3 = ¬(B·N1)/1, XOR (wzorzec)/2
  N1 = ¬(A·B)/1 -> N2 = ¬(A·N1)/2, N3 = ¬(B·N1)/2
  N2 = ¬(A·N1)/1 -> Y = ¬(N2·N3)/1
  N3 = ¬(B·N1)/1 -> Y = ¬(N2·N3)/2
  Y = ¬(N2·N3)/1 -> porównanie/1, Y/1
  XOR (wzorzec)/1 -> porównanie/2, Y_wz/1
  porównanie/1 -> XOR/1
